simulink model "hex_recovery"  (R2025b)
settings: Solver=FixedStepDiscrete  StartTime=0.0  StopTime=P.duration  FixedStep=P.base_dt  RelTol=1e-3
model workspace (MAT data in the model file):
  P.mass = 3.4
  P.gravity = 9.81
  P.rotor_positions = [0.275  0  0; 0.1375  0.238156986041  0; -0.1375  0.238156986041  0; -0.275  3.36777869766e-17  0; -0.1375  -0.238156986041  0; 0.1375  -0.238156986041  0]
  P.J = [0.0305275  -2.60208521397e-18  0; -2.60208521397e-18  0.0305275  0; 0  0  0.059375]
  P.invJ = [32.7573499304  2.79215185988e-15  0; 2.79215185988e-15  32.7573499304  0; 0  0  16.8421052632]
  P.kT = [7.45e-06; 7.45e-06; 7.45e-06; 7.45e-06; 7.45e-06; 7.45e-06]
  P.kQ = [9.79675e-08; 9.79675e-08; 9.79675e-08; 9.79675e-08; 9.79675e-08; 9.79675e-08]
  P.yaw_sign = [1; -1; 1; -1; 1; -1]
  P.tau = [0.05; 0.05; 0.05; 0.05; 0.05; 0.05]
  P.omega_min = 0
  P.omega_max = 1100
  P.body_drag = [0.005; 0.005; 0.01]
  P.rotor_drag = [0.000119; 0.000119; 0.000232]
  P.A = [1  1  1  1  1  1; 0  0.238156986041  0.238156986041  3.36777869766e-17  -0.238156986041  -0.238156986041; -0.275  -0.1375  0.1375  0.275  0.1375  -0.1375; 0.01315  -0.01315  0.01315  -0.01315  0.01315  -0.01315]
  P.pinvA = [0.166666666667  -3.00435841323e-17  -1.21212121212  12.6742712294; 0.166666666667  1.04972776216  -0.606060606061  -12.6742712294; 0.166666666667  1.04972776216  0.606060606061  12.6742712294; 0.166666666667  1.03568818436e-16  1.21212121212  -12.6742712294; 0.166666666667  -1.04972776216  0.606060606061  12.6742712294; 0.166666666667  -1.04972776216  -0.606060606061  -12.6742712294]
  P.thrust_min = [0; 0; 0; 0; 0; 0]
  P.thrust_max = [9.0145; 9.0145; 9.0145; 9.0145; 9.0145; 9.0145]
  P.wrench_scale = [54.087; 8.58746460266; 9.91595; 0.71124405]
  P.row_weights = [0.0369774622368; 0.116448806053; 0.100847624282; 0.281197431458]
  P.regularization = 0
  P.control.yaw_hold_rad = 0
  P.control.position_p = [4; 4; 1.4]
  P.control.velocity_p = [7; 7; 3]
  P.control.velocity_i = [0.4; 0.4; 0.9]
  P.control.velocity_d = [0.1; 0.1; 0.1]
  P.control.attitude_p = [7; 7; 3]
  P.control.rate_p = [20; 20; 6]
  P.control.rate_i = [30; 30; 0.6]
  P.control.rate_d = [0.5; 0.5; 0.06]
  P.control.velocity_limit_m_s = [3; 3; 2]
  P.control.rate_limit_rad_s = [3; 3; 1.5]
  P.control.velocity_integral_limit_m_s2 = [2; 2; 2]
  P.control.rate_integral_limit_rad_s2 = [20; 20; 2]
  P.control.acceleration_limit_m_s2 = [4; 4; 4]
  P.control.tilt_limit_deg = 25
  P.control.derivative_filter_hz = 20
  P.control.antiwindup_gain_s_inv = 2
  P.control.recovery.estimator_tau_s = 0.025
  P.control.recovery.estimator_min_command_rad_s = 100
  P.control.recovery.failed_speed_ratio = 0.06
  P.control.recovery.healthy_speed_ratio = 0.98
  P.control.recovery.position_soft_m = 0.08
  P.control.recovery.position_hard_m = 0.3
  P.control.recovery.tilt_soft_deg = 12
  P.control.recovery.tilt_hard_deg = 25
  P.control.recovery.rate_soft_rad_s = 0.6
  P.control.recovery.rate_hard_rad_s = 2
  P.control.recovery.progress_slow_tau_s = 0.08
  P.control.recovery.progress_fast_tau_s = 0.8
  P.control.recovery.degraded_position_p = [1.5; 1.5; 1.4]
  P.control.recovery.degraded_velocity_p = [4; 4; 3]
  P.control.recovery.degraded_acceleration_limit_m_s2 = [1.5; 1.5; 3]
  P.control.recovery.degraded_tilt_limit_deg = 15
  P.control.recovery.yaw_damping_s_inv = 1
  P.control.recovery.degraded_wrench_priority = [6; 3; 3; 0.015]
  P.sensor.rate_hz = 100
  P.sensor.accel_noise_density = 0.0035
  P.sensor.gyro_noise_density = 0.0003
  P.sensor.accel_bias_diffusion = 0.002
  P.sensor.gyro_bias_diffusion = 2e-05
  P.sensor.additional_accel_sample_std = 0.008
  P.sensor.position_sample_std_m = 0.003
  P.sensor.velocity_sample_std_m_s = 0.01
  P.sensor.attitude_sample_std_rad = 0.0008
  P.sensor.rpm_sample_std_rad_s = 1
  P.sensor.lever_m = [0; 0; 0]
  P.sensor.installation_rotation_xyzw = [0; 0; 0; 1]
  P.sensor.feedback_delay_s = 0.01
  P.sensor.installation_matrix = [1  0  0; 0  1  0; 0  0  1]
  P.wind.mean_m_s = [0; 0; 0]
  P.wind.ou_stationary_std_m_s = 0.2
  P.wind.ou_correlation_time_s = 1
  P.wind.update_rate_hz = 100
  P.termination.position_norm_m = 25
  P.termination.speed_m_s = 20
  P.termination.body_rate_rad_s = 15
  P.termination.minimum_altitude_m = -2
  P.integration_dt = 0.002
  P.control_dt = 0.01
  P.sensor_dt = 0.01
  P.export_dt = 0.01
  P.base_dt = 0.01
  P.duration = 24
  P.reference_mode = 'recovery_path_progress'
  P.control_tuning_version = 'recovery_v3_20261023'
  P.initial_state = [0; 0; 2.5; 0; 0; 0; 0; 0; 0; 1; 0; 0; 0; 863.81392478; 863.81392478; 863.81392478; 863.81392478; 863.81392478; 863.81392478]
  P.task_family = 2
  P.task_origin = [0; 0; 2.5]
  P.motion_start = 1
  P.motion_end = 7
  P.heading = 0
  P.displacement = 1.2
  P.radius = 0.3
  P.turn = 6.28318530718
  P.fault_motor = 1
  P.fault_factor = 0
  P.fault_start = 3
  P.fault_end = Inf
  P.observed_feedback = 1
  P.noise_enabled = 1
  P.wind_enabled = 1
  P.feedback_delay = 0.03
  P.seed = 20261006
  P.external_force = [0; 0; 0]
  P.external_torque = [0; 0; 0]
  P.exogenous = [-0.419748102169 -0.416018697024 -0.42343299448 -0.41045202828 -0.394392977316 -0.434544678836 -0.402415922967 -0.400265397714 -0.40478587178 -0.425441360189 -0.422504362468 -0.40174926008 ... (57648 elements, 2402x24)]
  P_controller_step.control.yaw_hold_rad = 0
  P_controller_step.control.position_p = [4; 4; 1.4]
  P_controller_step.control.velocity_p = [7; 7; 3]
  P_controller_step.control.velocity_i = [0.4; 0.4; 0.9]
  P_controller_step.control.velocity_d = [0.1; 0.1; 0.1]
  P_controller_step.control.attitude_p = [7; 7; 3]
  P_controller_step.control.rate_p = [20; 20; 6]
  P_controller_step.control.rate_i = [30; 30; 0.6]
  P_controller_step.control.rate_d = [0.5; 0.5; 0.06]
  P_controller_step.control.velocity_limit_m_s = [3; 3; 2]
  P_controller_step.control.rate_limit_rad_s = [3; 3; 1.5]
  P_controller_step.control.velocity_integral_limit_m_s2 = [2; 2; 2]
  P_controller_step.control.rate_integral_limit_rad_s2 = [20; 20; 2]
  P_controller_step.control.acceleration_limit_m_s2 = [4; 4; 4]
  P_controller_step.control.tilt_limit_deg = 25
  P_controller_step.control.derivative_filter_hz = 20
  P_controller_step.control.antiwindup_gain_s_inv = 2
  P_controller_step.control.recovery.estimator_tau_s = 0.025
  P_controller_step.control.recovery.estimator_min_command_rad_s = 100
  P_controller_step.control.recovery.failed_speed_ratio = 0.06
  P_controller_step.control.recovery.healthy_speed_ratio = 0.98
  P_controller_step.control.recovery.position_soft_m = 0.08
  P_controller_step.control.recovery.position_hard_m = 0.3
  P_controller_step.control.recovery.tilt_soft_deg = 12
  P_controller_step.control.recovery.tilt_hard_deg = 25
  P_controller_step.control.recovery.rate_soft_rad_s = 0.6
  P_controller_step.control.recovery.rate_hard_rad_s = 2
  P_controller_step.control.recovery.progress_slow_tau_s = 0.08
  P_controller_step.control.recovery.progress_fast_tau_s = 0.8
  P_controller_step.control.recovery.degraded_position_p = [1.5; 1.5; 1.4]
  P_controller_step.control.recovery.degraded_velocity_p = [4; 4; 3]
  P_controller_step.control.recovery.degraded_acceleration_limit_m_s2 = [1.5; 1.5; 3]
  P_controller_step.control.recovery.degraded_tilt_limit_deg = 15
  P_controller_step.control.recovery.yaw_damping_s_inv = 1
  P_controller_step.control.recovery.degraded_wrench_priority = [6; 3; 3; 0.015]
  P_controller_step.control_dt = 0.01
  P_controller_step.mass = 3.4
  P_controller_step.gravity = 9.81
  P_controller_step.thrust_max = [9.0145; 9.0145; 9.0145; 9.0145; 9.0145; 9.0145]
  P_controller_step.J = [0.0305275  -2.60208521397e-18  0; -2.60208521397e-18  0.0305275  0; 0  0  0.059375]
  P_controller_step.kT = [7.45e-06; 7.45e-06; 7.45e-06; 7.45e-06; 7.45e-06; 7.45e-06]
  P_controller_step.A = [1  1  1  1  1  1; 0  0.238156986041  0.238156986041  3.36777869766e-17  -0.238156986041  -0.238156986041; -0.275  -0.1375  0.1375  0.275  0.1375  -0.1375; 0.01315  -0.01315  0.01315  -0.01315  0.01315  -0.01315]
  P_controller_step.pinvA = [0.166666666667  -3.00435841323e-17  -1.21212121212  12.6742712294; 0.166666666667  1.04972776216  -0.606060606061  -12.6742712294; 0.166666666667  1.04972776216  0.606060606061  12.6742712294; 0.166666666667  1.03568818436e-16  1.21212121212  -12.6742712294; 0.166666666667  -1.04972776216  0.606060606061  12.6742712294; 0.166666666667  -1.04972776216  -0.606060606061  -12.6742712294]
  P_controller_step.thrust_min = [0; 0; 0; 0; 0; 0]
  P_controller_step.row_weights = [0.0369774622368; 0.116448806053; 0.100847624282; 0.281197431458]
  P_controller_step.wrench_scale = [54.087; 8.58746460266; 9.91595; 0.71124405]
  P_controller_step.regularization = 0
  P_controller_step.tau = [0.05; 0.05; 0.05; 0.05; 0.05; 0.05]
  P_controller_step.omega_max = 1100
  P_controller_step.observed_feedback = 1
  P_controller_step.feedback_delay = 0.03
  P_controller_step.sensor_dt = 0.01
  P_envelope_step.termination.position_norm_m = 25
  P_envelope_step.termination.speed_m_s = 20
  P_envelope_step.termination.body_rate_rad_s = 15
  P_envelope_step.termination.minimum_altitude_m = -2
  P_fault_schedule.base_dt = 0.01
  P_fault_schedule.fault_start = 3
  P_fault_schedule.fault_end = Inf
  P_fault_schedule.fault_motor = 1
  P_fault_schedule.fault_factor = 0
  P_plant_step.rotor_positions = [0.275  0  0; 0.1375  0.238156986041  0; -0.1375  0.238156986041  0; -0.275  3.36777869766e-17  0; -0.1375  -0.238156986041  0; 0.1375  -0.238156986041  0]
  P_plant_step.rotor_drag = [0.000119; 0.000119; 0.000232]
  P_plant_step.kT = [7.45e-06; 7.45e-06; 7.45e-06; 7.45e-06; 7.45e-06; 7.45e-06]
  P_plant_step.kQ = [9.79675e-08; 9.79675e-08; 9.79675e-08; 9.79675e-08; 9.79675e-08; 9.79675e-08]
  P_plant_step.yaw_sign = [1; -1; 1; -1; 1; -1]
  P_plant_step.body_drag = [0.005; 0.005; 0.01]
  P_plant_step.gravity = 9.81
  P_plant_step.mass = 3.4
  P_plant_step.invJ = [32.7573499304  2.79215185988e-15  0; 2.79215185988e-15  32.7573499304  0; 0  0  16.8421052632]
  P_plant_step.J = [0.0305275  -2.60208521397e-18  0; -2.60208521397e-18  0.0305275  0; 0  0  0.059375]
  P_plant_step.tau = [0.05; 0.05; 0.05; 0.05; 0.05; 0.05]
  P_plant_step.integration_dt = 0.002
  P_sensor_step.rotor_positions = [0.275  0  0; 0.1375  0.238156986041  0; -0.1375  0.238156986041  0; -0.275  3.36777869766e-17  0; -0.1375  -0.238156986041  0; 0.1375  -0.238156986041  0]
  P_sensor_step.rotor_drag = [0.000119; 0.000119; 0.000232]
  P_sensor_step.kT = [7.45e-06; 7.45e-06; 7.45e-06; 7.45e-06; 7.45e-06; 7.45e-06]
  P_sensor_step.kQ = [9.79675e-08; 9.79675e-08; 9.79675e-08; 9.79675e-08; 9.79675e-08; 9.79675e-08]
  P_sensor_step.yaw_sign = [1; -1; 1; -1; 1; -1]
  P_sensor_step.body_drag = [0.005; 0.005; 0.01]
  P_sensor_step.gravity = 9.81
  P_sensor_step.mass = 3.4
  P_sensor_step.invJ = [32.7573499304  2.79215185988e-15  0; 2.79215185988e-15  32.7573499304  0; 0  0  16.8421052632]
  P_sensor_step.J = [0.0305275  -2.60208521397e-18  0; -2.60208521397e-18  0.0305275  0; 0  0  0.059375]
  P_sensor_step.tau = [0.05; 0.05; 0.05; 0.05; 0.05; 0.05]
  P_sensor_step.sensor.rate_hz = 100
  P_sensor_step.sensor.accel_noise_density = 0.0035
  P_sensor_step.sensor.gyro_noise_density = 0.0003
  P_sensor_step.sensor.accel_bias_diffusion = 0.002
  P_sensor_step.sensor.gyro_bias_diffusion = 2e-05
  P_sensor_step.sensor.additional_accel_sample_std = 0.008
  P_sensor_step.sensor.position_sample_std_m = 0.003
  P_sensor_step.sensor.velocity_sample_std_m_s = 0.01
  P_sensor_step.sensor.attitude_sample_std_rad = 0.0008
  P_sensor_step.sensor.rpm_sample_std_rad_s = 1
  P_sensor_step.sensor.lever_m = [0; 0; 0]
  P_sensor_step.sensor.installation_rotation_xyzw = [0; 0; 0; 1]
  P_sensor_step.sensor.feedback_delay_s = 0.01
  P_sensor_step.sensor.installation_matrix = [1  0  0; 0  1  0; 0  0  1]
  P_sensor_step.sensor_dt = 0.01
  P_sensor_step.exogenous = [-0.419748102169 -0.416018697024 -0.42343299448 -0.41045202828 -0.394392977316 -0.434544678836 -0.402415922967 -0.400265397714 -0.40478587178 -0.425441360189 -0.422504362468 -0.40174926008 ... (57648 elements, 2402x24)]
  P_sensor_step.noise_enabled = 1
  P_sensor_step.observed_feedback = 1
  P_sensor_step.feedback_delay = 0.03
  P_task_reference.task_origin = [0; 0; 2.5]
  P_task_reference.task_family = 2
  P_task_reference.motion_start = 1
  P_task_reference.motion_end = 7
  P_task_reference.heading = 0
  P_task_reference.displacement = 1.2
  P_task_reference.radius = 0.3
  P_task_reference.turn = 6.28318530718
  P_task_reference.control.yaw_hold_rad = 0
  P_task_reference.control.position_p = [4; 4; 1.4]
  P_task_reference.control.velocity_p = [7; 7; 3]
  P_task_reference.control.velocity_i = [0.4; 0.4; 0.9]
  P_task_reference.control.velocity_d = [0.1; 0.1; 0.1]
  P_task_reference.control.attitude_p = [7; 7; 3]
  P_task_reference.control.rate_p = [20; 20; 6]
  P_task_reference.control.rate_i = [30; 30; 0.6]
  P_task_reference.control.rate_d = [0.5; 0.5; 0.06]
  P_task_reference.control.velocity_limit_m_s = [3; 3; 2]
  P_task_reference.control.rate_limit_rad_s = [3; 3; 1.5]
  P_task_reference.control.velocity_integral_limit_m_s2 = [2; 2; 2]
  P_task_reference.control.rate_integral_limit_rad_s2 = [20; 20; 2]
  P_task_reference.control.acceleration_limit_m_s2 = [4; 4; 4]
  P_task_reference.control.tilt_limit_deg = 25
  P_task_reference.control.derivative_filter_hz = 20
  P_task_reference.control.antiwindup_gain_s_inv = 2
  P_task_reference.control.recovery.estimator_tau_s = 0.025
  P_task_reference.control.recovery.estimator_min_command_rad_s = 100
  P_task_reference.control.recovery.failed_speed_ratio = 0.06
  P_task_reference.control.recovery.healthy_speed_ratio = 0.98
  P_task_reference.control.recovery.position_soft_m = 0.08
  P_task_reference.control.recovery.position_hard_m = 0.3
  P_task_reference.control.recovery.tilt_soft_deg = 12
  P_task_reference.control.recovery.tilt_hard_deg = 25
  P_task_reference.control.recovery.rate_soft_rad_s = 0.6
  P_task_reference.control.recovery.rate_hard_rad_s = 2
  P_task_reference.control.recovery.progress_slow_tau_s = 0.08
  P_task_reference.control.recovery.progress_fast_tau_s = 0.8
  P_task_reference.control.recovery.degraded_position_p = [1.5; 1.5; 1.4]
  P_task_reference.control.recovery.degraded_velocity_p = [4; 4; 3]
  P_task_reference.control.recovery.degraded_acceleration_limit_m_s2 = [1.5; 1.5; 3]
  P_task_reference.control.recovery.degraded_tilt_limit_deg = 15
  P_task_reference.control.recovery.yaw_damping_s_inv = 1
  P_task_reference.control.recovery.degraded_wrench_priority = [6; 3; 3; 0.015]
  P_task_reference.control_dt = 0.01
  P_wind_step.sensor_dt = 0.01
  P_wind_step.exogenous = [-0.419748102169 -0.416018697024 -0.42343299448 -0.41045202828 -0.394392977316 -0.434544678836 -0.402415922967 -0.400265397714 -0.40478587178 -0.425441360189 -0.422504362468 -0.40174926008 ... (57648 elements, 2402x24)]
  P_wind_step.wind_enabled = 1
  P_wind_step.external_force = [0; 0; 0]
  P_wind_step.external_torque = [0; 0; 0]
values from neighbouring files (symbols this model uses):
  P = hex_recovery_parameters(); ws.assignin('P',P)    [build_hex_recovery_model.m]    (also in diagnose_hex_healthy_tilt.m = base.parameters; hex_recovery_metrics.m = result.parameters; hex_recovery_parameters.m = hex_prepare_inputs(P); my_simulation.m = hex_prepare_inputs(P))
Description:
  | Six-rotor research simulation migrated from a6b9f1dd3d839416e469755490b8ff7733acd4ee. ENU world, FLU body, Hamilton xyzw, SI units. Embedded MATLAB Function code; no Python runtime. 100 Hz controller/sensors, 500 Hz RK4 substeps; fault truth enters plant only.
  | 
  | # SciPy trust-region-reflective algorithm
  | 
  | `functions/hex_trf.m` is a MATLAB translation/adaptation of the bounded linear least-squares algorithm in SciPy 1.17.1:
  | 
  | - `scipy/optimize/_lsq/trf_linear.py`
  | - `scipy/optimize/_lsq/common.py` (bounded-linear-solver helpers)
  | - `scipy/optimize/_lsq/givens_elimination.pyx`
  | 
  | Source: https://github.com/scipy/scipy/tree/v1.17.1/scipy/optimize/_lsq
  | 
  | The implementation is restricted to six variables with finite bounds and uses MATLAB's QR/SVD kernels. It is embedded in the delivered SLX; the upstream Python runtime and SciPy binaries are not required for simulation.
  | 
  | ```text
  | Copyright (c) 2001-2002 Enthought, Inc. 2003, SciPy Developers.
  | All rights reserved.
  | 
  | Redistribution and use in source and binary forms, with or without
  | modification, are permitted provided that the following conditions
  | are met:
  | 
  | 1. Redistributions of source code must retain the above copyright
  |    notice, this list of conditions and the following disclaimer.
  | 
  | 2. Redistributions in binary form must reproduce the above
  |    copyright notice, this list of conditions and the following
  |    disclaimer in the documentation and/or other materials provided
  |    with the distribution.
  | 
  | 3. Neither the name of the copyright holder nor the names of its
  |    contributors may be used to endorse or promote products derived
  |    from this software without specific prior written permission.
  | 
  | THIS SOFTWARE IS PROVIDED BY THE COPYRIGHT HOLDERS AND CONTRIBUTORS
  | "AS IS" AND ANY EXPRESS OR IMPLIED WARRANTIES, INCLUDING, BUT NOT
  | LIMITED TO, THE IMPLIED WARRANTIES OF MERCHANTABILITY AND FITNESS FOR
  | A PARTICULAR PURPOSE ARE DISCLAIMED. IN NO EVENT SHALL THE COPYRIGHT
  | OWNER OR CONTRIBUTORS BE LIABLE FOR ANY DIRECT, INDIRECT, INCIDENTAL,
  | SPECIAL, EXEMPLARY, OR CONSEQUENTIAL DAMAGES (INCLUDING, BUT NOT
  | LIMITED TO, PROCUREMENT OF SUBSTITUTE GOODS OR SERVICES; LOSS OF USE,
  | DATA, OR PROFITS; OR BUSINESS INTERRUPTION) HOWEVER CAUSED AND ON ANY
  | THEORY OF LIABILITY, WHETHER IN CONTRACT, STRICT LIABILITY, OR TORT
  | (INCLUDING NEGLIGENCE OR OTHERWISE) ARISING IN ANY WAY OUT OF THE USE
  | OF THIS SOFTWARE, EVEN IF ADVISED OF THE POSSIBILITY OF SUCH DAMAGE.
  | ```
  | 
  | 
  | Copyright 2023 RotorPy Authors
  | 
  | Permission is hereby granted, free of charge, to any person obtaining a copy of this software and associated documentation files (the "Software"), to deal in the Software without restriction, including without limitation the rights to use, copy, modify, merge, publish, distribute, sublicense, and/or sell copies of the Software, and to permit persons to whom the Software is furnished to do so, subject to the following conditions:
  | 
  | The above copyright notice and this permission notice shall be included in all copies or substantial portions of the Software.
  | 
  | THE SOFTWARE IS PROVIDED "AS IS", WITHOUT WARRANTY OF ANY KIND, EXPRESS OR IMPLIED, INCLUDING BUT NOT LIMITED TO THE WARRANTIES OF MERCHANTABILITY, FITNESS FOR A PARTICULAR PURPOSE AND NONINFRINGEMENT. IN NO EVENT SHALL THE AUTHORS OR COPYRIGHT HOLDERS BE LIABLE FOR ANY CLAIM, DAMAGES OR OTHER LIABILITY, WHETHER IN AN ACTION OF CONTRACT, TORT OR OTHERWISE, ARISING FROM, OUT OF OR IN CONNECTION WITH THE SOFTWARE OR THE USE OR OTHER DEALINGS IN THE SOFTWARE.
  | 
  | PV reference: position/velocity only; internal fixed heading; no acceleration or yaw-rate feedforward.
  | Recovery experiment 2026-10-23: RPM-based estimate; thrust-direction priority; measured-state path retiming.
settings Model: Creator=lenovo  LastModifiedBy=lenovo
settings DataIOCC: SaveOutput=off  SignalLogging=off

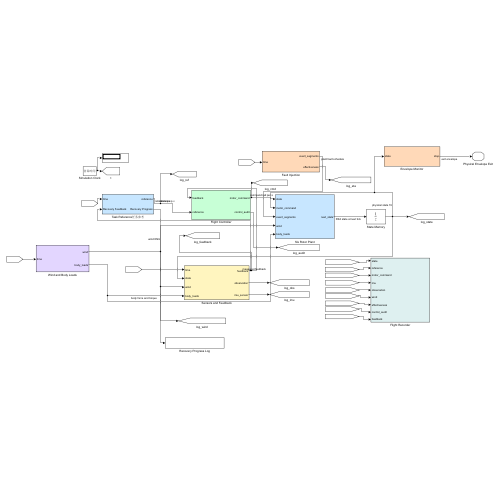
[thumbnail: Simulink's stored preview of the top-level diagram]
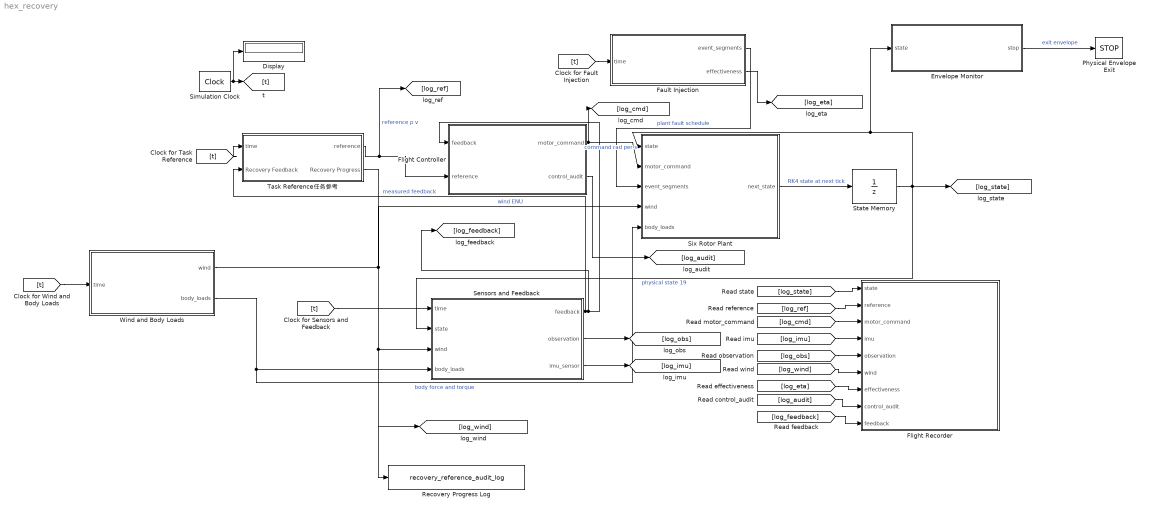
== system hex_recovery ==
  Display : Display
  Envelope Monitor : Subsystem
  Fault Injection : Subsystem
  Flight Controller : Subsystem
  Flight Recorder : Subsystem
  Physical Envelope Exit : Stop
  Recovery Progress Log : ToWorkspace  VariableName=recovery_reference_audit_log  SaveFormat=Timeseries  SampleTime=P.export_dt
  Sensors and Feedback : Subsystem
  Simulation Clock : DigitalClock  SampleTime=P.base_dt
      mask DialogControl ParameterGroupVar Prompt: 参数
      mask Display: disp('仿真时间')
  Six Rotor Plant : Subsystem
  State Memory : UnitDelay  InitialCondition=P.initial_state  SampleTime=P.base_dt  HasFrameUpgradeWarning=on
  Task Reference任务参考 : Subsystem
  Wind and Body Loads : Subsystem
  wires:
  Simulation Clock/1 -> Display/1, [t]
  [t] -> Task Reference任务参考/1(time)
  [t] -> Fault Injection/1(time)
  [t] -> Wind and Body Loads/1(time)
  [t] -> Sensors and Feedback/1(time)
  Task Reference任务参考/1(reference) -> Flight Controller/2(reference), [log_ref]  "reference p v"
  Sensors and Feedback/1(feedback) -> Flight Controller/1(feedback), [log_feedback], Task Reference任务参考/2(Recovery Feedback)  "measured feedback"
  Flight Controller/1(motor_command) -> Six Rotor Plant/2(motor_command), [log_cmd]  "command rad per s"
  Fault Injection/1(event_segments) -> Six Rotor Plant/3(event_segments)  "plant fault schedule"
  Wind and Body Loads/1(wind) -> Sensors and Feedback/3(wind), [log_wind], Six Rotor Plant/4(wind)  "wind ENU"
  Wind and Body Loads/2(body_loads) -> Sensors and Feedback/4(body_loads), Six Rotor Plant/5(body_loads)  "body force and torque"
  Six Rotor Plant/1(next_state) -> State Memory/1  "RK4 state at next tick"
  State Memory/1 -> Six Rotor Plant/1(state), Envelope Monitor/1(state), [log_state], Sensors and Feedback/2(state)  "physical state 19"
  Envelope Monitor/1(stop) -> Physical Envelope Exit/1  "exit envelope"
  [log_state] -> Flight Recorder/1(state)
  [log_ref] -> Flight Recorder/2(reference)
  [log_cmd] -> Flight Recorder/3(motor_command)
  Sensors and Feedback/3(imu_sensor) -> [log_imu]
  [log_imu] -> Flight Recorder/4(imu)
  Sensors and Feedback/2(observation) -> [log_obs]
  [log_obs] -> Flight Recorder/5(observation)
  [log_wind] -> Flight Recorder/6(wind)
  Fault Injection/2(effectiveness) -> [log_eta]
  [log_eta] -> Flight Recorder/7(effectiveness)
  Flight Controller/2(control_audit) -> [log_audit]
  [log_audit] -> Flight Recorder/8(control_audit)
  [log_feedback] -> Flight Recorder/9(feedback)
  Task Reference任务参考/2(Recovery Progress) -> Recovery Progress Log/1

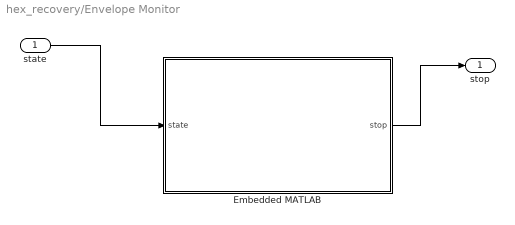
== system hex_recovery/Envelope Monitor ==
  state : Inport
  Embedded MATLAB : MATLAB Function  TreatAsAtomicUnit=on
  stop : Outport
  wires:
  state/1 -> Embedded MATLAB/1(state)
  Embedded MATLAB/1(stop) -> stop/1

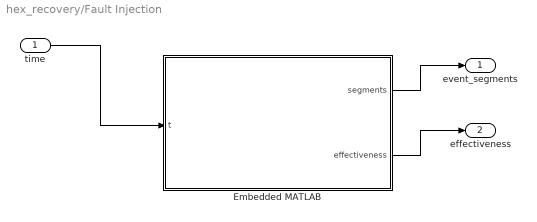
== system hex_recovery/Fault Injection ==
  time : Inport
  Embedded MATLAB : MATLAB Function  TreatAsAtomicUnit=on
  event_segments : Outport
  effectiveness : Outport  Port=2
  wires:
  time/1 -> Embedded MATLAB/1(t)
  Embedded MATLAB/1(segments) -> event_segments/1
  Embedded MATLAB/2(effectiveness) -> effectiveness/1

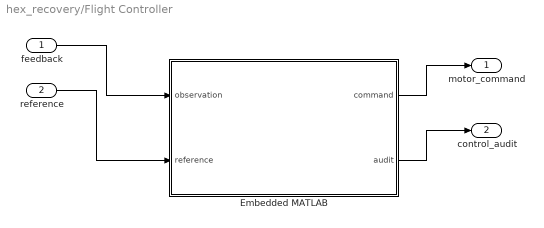
== system hex_recovery/Flight Controller ==
  feedback : Inport
  reference : Inport  Port=2
  Embedded MATLAB : MATLAB Function  TreatAsAtomicUnit=on
  motor_command : Outport
  control_audit : Outport  Port=2
  wires:
  feedback/1 -> Embedded MATLAB/1(observation)
  reference/1 -> Embedded MATLAB/2(reference)
  Embedded MATLAB/1(command) -> motor_command/1
  Embedded MATLAB/2(audit) -> control_audit/1

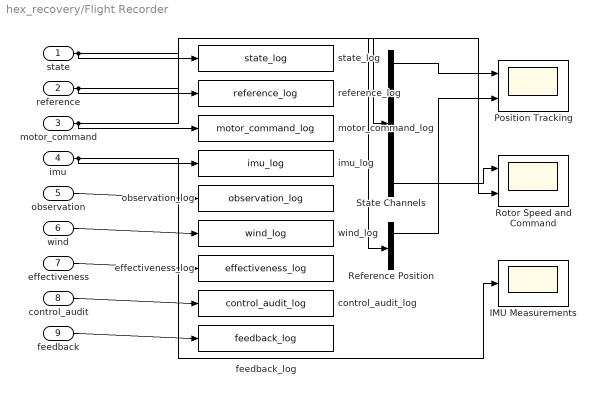
== system hex_recovery/Flight Recorder ==
  state : Inport
  reference : Inport  Port=2
  motor_command : Inport  Port=3
  imu : Inport  Port=4
  observation : Inport  Port=5
  wind : Inport  Port=6
  effectiveness : Inport  Port=7
  control_audit : Inport  Port=8
  feedback : Inport  Port=9
  IMU Measurements : Scope
  Position Tracking : Scope  NumInputPorts=2
  Reference Position : Demux  Outputs=[3 3]
  Rotor Speed and Command : Scope  NumInputPorts=2
  State Channels : Demux  Outputs=[3 3 4 3 6]
  control_audit_log : ToWorkspace  VariableName=control_audit_log  SaveFormat=Timeseries  SampleTime=P.export_dt
  effectiveness_log : ToWorkspace  VariableName=effectiveness_log  SaveFormat=Timeseries  SampleTime=P.export_dt
  feedback_log : ToWorkspace  VariableName=feedback_log  SaveFormat=Timeseries  SampleTime=P.export_dt
  imu_log : ToWorkspace  VariableName=imu_log  SaveFormat=Timeseries  SampleTime=P.export_dt
  motor_command_log : ToWorkspace  VariableName=motor_command_log  SaveFormat=Timeseries  SampleTime=P.export_dt
  observation_log : ToWorkspace  VariableName=observation_log  SaveFormat=Timeseries  SampleTime=P.export_dt
  reference_log : ToWorkspace  VariableName=reference_log  SaveFormat=Timeseries  SampleTime=P.export_dt
  state_log : ToWorkspace  VariableName=state_log  SaveFormat=Timeseries  SampleTime=P.export_dt
  wind_log : ToWorkspace  VariableName=wind_log  SaveFormat=Timeseries  SampleTime=P.export_dt
  wires:
  state/1 -> state_log/1, State Channels/1
  reference/1 -> reference_log/1, Reference Position/1
  motor_command/1 -> motor_command_log/1, Rotor Speed and Command/2
  imu/1 -> imu_log/1, IMU Measurements/1
  observation/1 -> observation_log/1
  wind/1 -> wind_log/1
  effectiveness/1 -> effectiveness_log/1
  control_audit/1 -> control_audit_log/1
  feedback/1 -> feedback_log/1
  State Channels/1 -> Position Tracking/1
  Reference Position/1 -> Position Tracking/2
  State Channels/5 -> Rotor Speed and Command/1

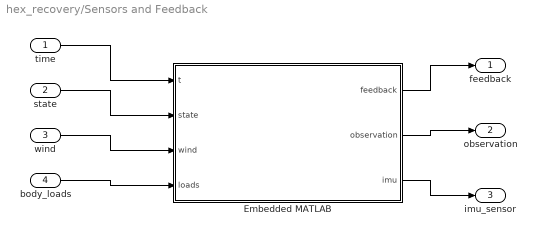
== system hex_recovery/Sensors and Feedback ==
  time : Inport
  state : Inport  Port=2
  wind : Inport  Port=3
  body_loads : Inport  Port=4
  Embedded MATLAB : MATLAB Function  TreatAsAtomicUnit=on
  feedback : Outport
  observation : Outport  Port=2
  imu_sensor : Outport  Port=3
  wires:
  time/1 -> Embedded MATLAB/1(t)
  state/1 -> Embedded MATLAB/2(state)
  wind/1 -> Embedded MATLAB/3(wind)
  body_loads/1 -> Embedded MATLAB/4(loads)
  Embedded MATLAB/1(feedback) -> feedback/1
  Embedded MATLAB/2(observation) -> observation/1
  Embedded MATLAB/3(imu) -> imu_sensor/1

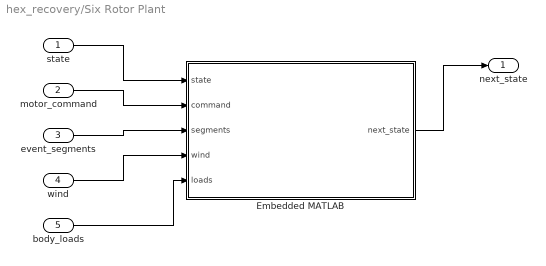
== system hex_recovery/Six Rotor Plant ==
  state : Inport
  motor_command : Inport  Port=2
  event_segments : Inport  Port=3
  wind : Inport  Port=4
  body_loads : Inport  Port=5
  Embedded MATLAB : MATLAB Function  TreatAsAtomicUnit=on
  next_state : Outport
  wires:
  state/1 -> Embedded MATLAB/1(state)
  motor_command/1 -> Embedded MATLAB/2(command)
  event_segments/1 -> Embedded MATLAB/3(segments)
  wind/1 -> Embedded MATLAB/4(wind)
  body_loads/1 -> Embedded MATLAB/5(loads)
  Embedded MATLAB/1(next_state) -> next_state/1

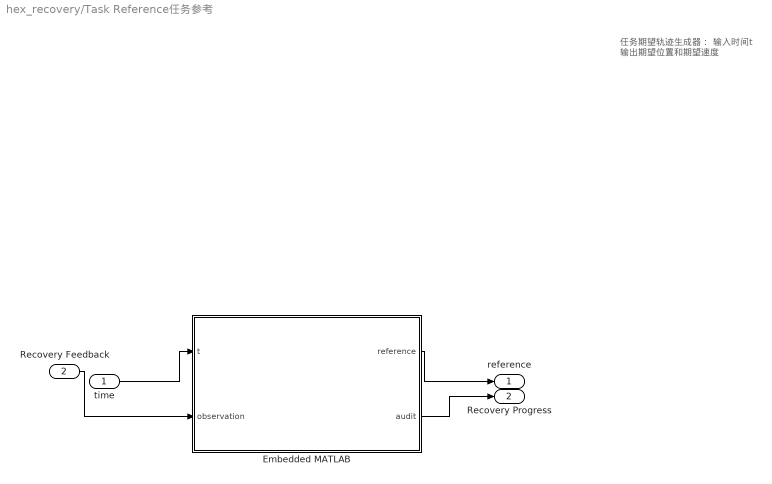
== system hex_recovery/Task Reference任务参考 ==
  note: 任务期望轨迹生成器：
      | 输入时间t
      | 输出期望位置和期望速度
  time : Inport
  Recovery Feedback : Inport  Port=2
  Embedded MATLAB : MATLAB Function  TreatAsAtomicUnit=on
  reference : Outport
  Recovery Progress : Outport  Port=2
  wires:
  time/1 -> Embedded MATLAB/1(t)
  Embedded MATLAB/1(reference) -> reference/1
  Recovery Feedback/1 -> Embedded MATLAB/2(observation)
  Embedded MATLAB/2(audit) -> Recovery Progress/1

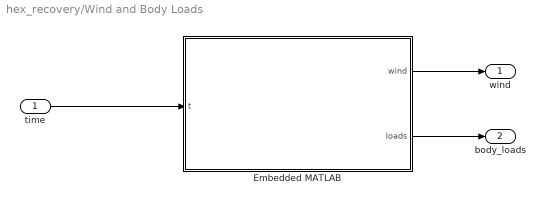
== system hex_recovery/Wind and Body Loads ==
  time : Inport
  Embedded MATLAB : MATLAB Function  TreatAsAtomicUnit=on
  wind : Outport
  body_loads : Outport  Port=2
  wires:
  time/1 -> Embedded MATLAB/1(t)
  Embedded MATLAB/1(wind) -> wind/1
  Embedded MATLAB/2(loads) -> body_loads/1

== matlab function hex_recovery/Flight Controller/Embedded MATLAB ==
  settings: updateMethod=DISCRETE  sampleTime=P.control_dt
  data: observation input; command output; reference input; audit output; P_controller_step parameter
function [command,audit]=recovery_controller_step(observation,reference,P_controller_step)
%#codegen
% Motor response is estimated from RPM feedback and delayed command history.
% Fault truth is not an input. eta_hat describes command-to-thrust loss only
% for this project's first-order motor-target failure model.
persistent previous_w previous_v filtered_alpha filtered_accel vi ri last_qd
persistent previous_rpm speed_ratio command_history ticks initialized
if isempty(initialized)
    previous_w=zeros(3,1); previous_v=zeros(3,1);
    filtered_alpha=zeros(3,1); filtered_accel=zeros(3,1);
    vi=zeros(3,1); ri=zeros(3,1); last_qd=[0;0;0;1];
    previous_rpm=zeros(6,1); speed_ratio=ones(6,1);
    command_history=zeros(6,1001); ticks=0; initialized=false;
end
x=observation(1:3); v=observation(4:6);
q=observation(7:10); q=q/norm(q); w=observation(11:13);
rpm=observation(14:19); R=hex_rotation(q);
c=P_controller_step.control; r=c.recovery; dt=P_controller_step.control_dt;
delay_ticks=0;
if P_controller_step.observed_feedback, delay_ticks=ceil(P_controller_step.feedback_delay/P_controller_step.sensor_dt-1e-10); end
if initialized && ticks>delay_ticks
    previous_command=command_history(:,mod(ticks-delay_ticks-1,1001)+1);
    decay=exp(-dt./P_controller_step.tau);
    for i=1:6
        if previous_command(i)>=r.estimator_min_command_rad_s
            observed=(rpm(i)-decay(i)*previous_rpm(i))/...
                ((1-decay(i))*previous_command(i));
            observed=min(max(observed,0),1.1);
            speed_ratio(i)=speed_ratio(i)+(1-exp(-dt/r.estimator_tau_s))*(observed-speed_ratio(i));
        end
    end
end
eta=min(speed_ratio.^2,1);
eta(speed_ratio>=r.healthy_speed_ratio)=1;
eta(speed_ratio<r.failed_speed_ratio)=0;
damage=min(max((1-min(eta))/.8,0),1);
position_p=(1-damage)*c.position_p+damage*r.degraded_position_p;
velocity_p=(1-damage)*c.velocity_p+damage*r.degraded_velocity_p;
acc_limit=(1-damage)*c.acceleration_limit_m_s2+damage*r.degraded_acceleration_limit_m_s2;
tilt_limit=(1-damage)*c.tilt_limit_deg+damage*r.degraded_tilt_limit_deg;
vi_applied=vi; ri_applied=ri;
ev=min(max(reference(4:6)+position_p.*(reference(1:3)-x),...
    -c.velocity_limit_m_s),c.velocity_limit_m_s)-v;
filt=1-exp(-2*pi*c.derivative_filter_hz*dt);
if initialized
    filtered_alpha=filtered_alpha+filt*((w-previous_w)/dt-filtered_alpha);
    filtered_accel=filtered_accel+filt*((v-previous_v)/dt-filtered_accel);
end
a_raw=velocity_p.*ev+vi-c.velocity_d.*filtered_accel;
acc=min(max(a_raw,-acc_limit),acc_limit);
F=P_controller_step.mass*(acc+[0;0;P_controller_step.gravity]); F(3)=max(F(3),0);
max_horizontal=F(3)*tan(tilt_limit*pi/180);
if norm(F(1:2))>max_horizontal
    F(1:2)=F(1:2)*max_horizontal/max(norm(F(1:2)),1e-12);
end
maximum=sum(eta.*P_controller_step.thrust_max);
if norm(F)>maximum, F=F*maximum/max(norm(F),1e-12); end
qd=hex_desired_attitude(F,c.yaw_hold_rad,last_qd);
e=hex_multiply([-q(1:3);q(4)],qd);
sgn=1; if e(4)<0, sgn=-1; end
attitude_error=2*sgn*e(1:3);
if damage>.1
    % Thrust direction has priority over heading during degraded flight.
    attitude_error=R'*cross(R(:,3),F/max(norm(F),1e-12));
end
rates=min(max(c.attitude_p.*attitude_error,-c.rate_limit_rad_s),c.rate_limit_rad_s);
error=rates-w;
alpha=c.rate_p.*error+ri-c.rate_d.*filtered_alpha;
if damage>.1
    rates(3)=0; error(3)=-w(3);
    alpha(3)=-r.yaw_damping_s_inv*w(3); ri(3)=0;
end
moment=P_controller_step.J*alpha+cross(w,P_controller_step.J*w);
desired=[max(F'*R(:,3),0);moment];
Q=P_controller_step; Q.thrust_max=max(eta.*P_controller_step.thrust_max,1e-9);
Q.thrust_min=zeros(6,1);
if damage>.1, Q.row_weights=r.degraded_wrench_priority./P_controller_step.wrench_scale; end
[thrust,residual,flags]=hex_allocate(desired,Q);
thrust=min(thrust,eta.*P_controller_step.thrust_max);
di=c.rate_i.*error*dt; di((residual(2:4).*error)>1e-8)=0;
if damage>.1, di(3)=0; end
ri=min(max(ri+di,-c.rate_integral_limit_rad_s2),c.rate_integral_limit_rad_s2);
limited_acc=F/P_controller_step.mass-[0;0;P_controller_step.gravity]; direction=F/max(norm(F),1e-12);
vi=min(max(vi+dt*(c.velocity_i.*ev+c.antiwindup_gain_s_inv*...
    (limited_acc-a_raw-direction*residual(1)/P_controller_step.mass)),...
    -c.velocity_integral_limit_m_s2),c.velocity_integral_limit_m_s2);
command=min(sqrt(max(thrust,0)./P_controller_step.kT)./max(sqrt(eta),1e-8),P_controller_step.omega_max);
command(eta==0)=0;
audit=[desired;P_controller_step.A*thrust;residual;vi;ri;reference(1:3)-x;ev;error;qd;rates;flags;...
    vi_applied;ri_applied;eta;damage];
command_history(:,mod(ticks,1001)+1)=command;
previous_rpm=rpm; previous_w=w; previous_v=v; last_qd=qd;
ticks=ticks+1; initialized=true;
end

function R=hex_rotation(q)
q=q/norm(q); v=q(1:3); w=q(4);
S=[0 -v(3) v(2);v(3) 0 -v(1);-v(2) v(1) 0];
R=eye(3)+2*w*S+2*S*S;
end

function q=hex_multiply(a,b)
q=[a(4)*b(1:3)+b(4)*a(1:3)+cross(a(1:3),b(1:3));a(4)*b(4)-a(1:3)'*b(1:3)];
end

function q=hex_desired_attitude(F,yaw,previous)
if norm(F)<1e-10
    q=previous/norm(previous); return
end
z=F/norm(F); y=cross(z,[cos(yaw);sin(yaw);0]);
if norm(y)<1e-10
    [~,i]=min(abs(z)); basis=zeros(3,1); basis(i)=1; y=cross(z,basis);
end
y=y/norm(y); x=cross(y,z); R=[x,y,z];
% Hamilton xyzw; branch on the largest component for numerical stability.
choices=[R(1,1);R(2,2);R(3,3);trace(R)]; [~,i]=max(choices);
if i==4
    w=sqrt(max(0,1+trace(R)))/2;
    q=[(R(3,2)-R(2,3))/(4*w);(R(1,3)-R(3,1))/(4*w);(R(2,1)-R(1,2))/(4*w);w];
else
    j=mod(i,3)+1; k=mod(j,3)+1;
    q=zeros(4,1); q(i)=sqrt(max(0,1+R(i,i)-R(j,j)-R(k,k)))/2;
    q(j)=(R(j,i)+R(i,j))/(4*q(i)); q(k)=(R(k,i)+R(i,k))/(4*q(i));
    q(4)=(R(k,j)-R(j,k))/(4*q(i));
end
q=q/norm(q);
end

function [thrust,residual,flags]=hex_allocate(desired,P_controller_step)
candidate=P_controller_step.pinvA*desired;
if P_controller_step.regularization==0 && all(candidate>=P_controller_step.thrust_min-1e-8) && all(candidate<=P_controller_step.thrust_max+1e-8) && norm(P_controller_step.row_weights.*(desired-P_controller_step.A*candidate))<=1e-10
    thrust=min(max(candidate,P_controller_step.thrust_min),P_controller_step.thrust_max); success=true;
else
    weights=diag(P_controller_step.row_weights);
    C=[weights*P_controller_step.A;sqrt(P_controller_step.regularization)*diag(1./max(P_controller_step.thrust_max-P_controller_step.thrust_min,1e-12))];
    d=[weights*desired;zeros(6,1)];
    [thrust,exitflag]=hex_trf(C,d,P_controller_step.thrust_min,P_controller_step.thrust_max);
    thrust=min(max(thrust,P_controller_step.thrust_min),P_controller_step.thrust_max);
    % A rank-deficient six-actuator problem can return a nonpositive flag
    % after reaching its optimum. Independently verify convex box KKT terms.
    gradient=C'*(C*thrust-d);
    projected=gradient;
    at_lower=thrust<=P_controller_step.thrust_min+1e-8;
    at_upper=thrust>=P_controller_step.thrust_max-1e-8;
    projected(at_lower)=min(gradient(at_lower),0);
    projected(at_upper)=max(gradient(at_upper),0);
    success=all(isfinite(thrust)) && (exitflag>0 || norm(projected,Inf)<=1e-10);
    if ~success
        fprintf('ALLOCATION_FAILURE flag=%g kkt=%.17g desired=[%.17g %.17g %.17g %.17g]\n',exitflag,norm(projected,Inf),desired(1),desired(2),desired(3),desired(4));
    end
end
residual=desired-P_controller_step.A*thrust;
boundtol=max(1e-8,1e-7*max(1,P_controller_step.thrust_max-P_controller_step.thrust_min));
active=(abs(thrust-P_controller_step.thrust_min)<=boundtol)|(abs(thrust-P_controller_step.thrust_max)<=boundtol);
flags=[double(success);sum(active);double(max(abs(residual./P_controller_step.wrench_scale))<=1e-6)];
assert(success,'Nominal allocation failed to converge.');
end

function [x,status]=hex_trf(A,b,lb,ub)
%HEX_TRF Six-variable trust-region-reflective bounded linear least squares.
% Algorithm translated from scipy.optimize._lsq.trf_linear/common, SciPy
% 1.17.1 (BSD-3-Clause; see THIRD_PARTY_NOTICES.md).
tol=1e-10;
QT=zeros(6,10); Rbase=zeros(6,6);
if all(A(5:10,:)==0,'all')
    x=pinv(A(1:4,:))*b(1:4);
    [Qsmall,Rsmall,E]=qr(A(1:4,:));
    QT(1:4,1:4)=Qsmall'; Rbase(1:4,:)=Rsmall;
else
    x=pinv(A)*b;
    [Qfull,Rfull,E]=qr(A,'econ'); QT=Qfull'; Rbase=Rfull;
end
[~,permutation]=max(E,[],1);
if all(x>=lb) && all(x<=ub), status=3; return; end
x=interior(reflect(x,lb,ub),lb,ub,.1);
r=A*x-b; g=A'*r; cost=.5*(r'*r); status=0;
for iteration=1:200
    v=ones(6,1); dv=zeros(6,1);
    for j=1:6
        if g(j)<0, v(j)=ub(j)-x(j); dv(j)=-1;
        elseif g(j)>0, v(j)=x(j)-lb(j); dv(j)=1;
        end
    end
    gnorm=norm(g.*v,Inf);
    if gnorm<tol, status=1; end
    if status~=0, break; end
    h=g.*dv; d=sqrt(v); gh=d.*g; Ah=A.*d';
    ph=-regularized_qr(Rbase.*d(permutation)',QT*r,permutation,sqrt(h));
    p=d.*ph; pg=p'*g;
    if pg>0, status=-1; end
    theta=1-min(.005,gnorm);
    step=select_step(x,Ah,gh,h,p,ph,d,lb,ub,theta);
    change=-quadratic(A,g,step,zeros(6,1));
    if change<0
        alpha=1;
        for backtrack=1:100
            xn=reflect(x+alpha*p,lb,ub); step=xn-x;
            change=-quadratic(A,g,step,zeros(6,1));
            if change>-.1*alpha*pg, break; end
            alpha=alpha*.5;
        end
        if any(active_bounds(xn,lb,ub,1e-10)~=0)
            xn=interior(reflect(x+theta*alpha*p,lb,ub),lb,ub,0);
            step=xn-x; change=-quadratic(A,g,step,zeros(6,1));
        end
        % Preserve the upstream backtracking routine's returned x exactly.
    else
        x=interior(x+step,lb,ub,0);
    end
    r=A*x-b; g=A'*r;
    if change<tol*cost, status=2; end
    cost=.5*(r'*r);
end
end

function x=regularized_qr(R,rhs,permutation,diagonal)
diagonal=diagonal(permutation);
for i=1:6
    if diagonal(i)==0, continue; end
    row=zeros(6,1); row(i)=diagonal(i); u=0;
    for j=i:6
        if row(j)~=0
            f=R(j,j); g=row(j);
            if f==0
                cs=0; sn=sign(g); radius=abs(g);
            else
                radius=sign(f)*hypot(f,g); cs=f/radius; sn=g/radius;
            end
            R(j,j)=radius;
            for k=j+1:6
                old=R(j,k); R(j,k)=cs*old+sn*row(k); row(k)=-sn*old+cs*row(k);
            end
            old=rhs(j); rhs(j)=cs*old+sn*u; u=-sn*old+cs*u;
        end
    end
end
valid=abs(diag(R))>eps*10*max(abs(diag(R)));
z=zeros(6,1);
for j=6:-1:1
    if valid(j)
        value=rhs(j);
        for k=j+1:6
            if valid(k), value=value-R(j,k)*z(k); end
        end
        z(j)=value/R(j,j);
    end
end
x=zeros(6,1);
for j=1:6, x(permutation(j))=z(j); end
end

function step=select_step(x,A,g,h,p,ph,d,lb,ub,theta)
if all(x+p>=lb) && all(x+p<=ub), step=p; return; end
[stride,hits]=bound_stride(x,p,lb,ub);
rh=ph; rh(hits)=-rh(hits); reflected=d.*rh;
p=p*stride; ph=ph*stride; on_bound=x+p;
[upper,~]=bound_stride(on_bound,reflected,lb,ub);
lower=(1-theta)*upper; upper=theta*upper;
rvalue=Inf;
if upper>0
    [a,b,c]=line_quadratic(A,g,h,rh,ph);
    [stride,rvalue]=min_line(a,b,c,lower,upper);
    rh=ph+rh*stride; reflected=d.*rh;
end
p=p*theta; ph=ph*theta;
pvalue=quadratic(A,g,ph,h);
agh=-g; ag=d.*agh;
[upper,~]=bound_stride(x,ag,lb,ub); upper=theta*upper;
[a,b,~]=line_quadratic(A,g,h,agh,zeros(6,1));
[stride,agvalue]=min_line(a,b,0,0,upper); ag=ag*stride;
if pvalue<rvalue && pvalue<agvalue, step=p;
elseif rvalue<pvalue && rvalue<agvalue, step=reflected;
else, step=ag;
end
end

function x=reflect(y,lb,ub)
x=y;
if all(y>=lb) && all(y<=ub), return; end
width=ub-lb; z=mod(y-lb,2*width);
x=lb+min(z,2*width-z);
end

function mask=active_bounds(x,lb,ub,tol)
mask=zeros(6,1);
for j=1:6
    if tol==0
        if x(j)<=lb(j), mask(j)=-1; end
        if x(j)>=ub(j), mask(j)=1; end
    else
        lower=x(j)-lb(j); upper=ub(j)-x(j);
        if lower<=min(upper,tol*max(1,abs(lb(j)))), mask(j)=-1; end
        if upper<=min(lower,tol*max(1,abs(ub(j)))), mask(j)=1; end
    end
end
end

function x=interior(x,lb,ub,relative_step)
mask=active_bounds(x,lb,ub,relative_step);
for j=1:6
    if mask(j)==-1
        if relative_step==0, x(j)=lb(j)+eps(lb(j));
        else, x(j)=lb(j)+relative_step*max(1,abs(lb(j))); end
    elseif mask(j)==1
        if relative_step==0, x(j)=ub(j)-eps(ub(j));
        else, x(j)=ub(j)-relative_step*max(1,abs(ub(j))); end
    end
    if x(j)<lb(j) || x(j)>ub(j), x(j)=(lb(j)+ub(j))/2; end
end
end

function [stride,hits]=bound_stride(x,s,lb,ub)
steps=Inf(6,1);
for j=1:6
    if s(j)~=0, steps(j)=max((lb(j)-x(j))/s(j),(ub(j)-x(j))/s(j)); end
end
stride=min(steps); hits=steps==stride;
end

function value=quadratic(A,g,s,h)
v=A*s; value=.5*(v'*v+(s.*h)'*s)+g'*s;
end

function [a,b,c]=line_quadratic(A,g,h,s,s0)
v=A*s; u=A*s0;
a=.5*(v'*v+(s.*h)'*s);
b=g'*s+u'*v+(s0.*h)'*s;
c=.5*(u'*u)+g'*s0+.5*(s0.*h)'*s0;
end

function [t,value]=min_line(a,b,c,lb,ub)
t=lb; value=lb*(a*lb+b)+c;
upper_value=ub*(a*ub+b)+c;
if upper_value<value, t=ub; value=upper_value; end
if a~=0
    stationary=-.5*b/a;
    if stationary>lb && stationary<ub
        stationary_value=stationary*(a*stationary+b)+c;
        if stationary_value<value, t=stationary; value=stationary_value; end
    end
end
end

== matlab function hex_recovery/Task Reference任务参考/Embedded MATLAB ==
  settings: updateMethod=DISCRETE  sampleTime=P.control_dt
  data: t input; observation input; reference output; P_task_reference parameter; audit output
function [reference,audit]=recovery_reference_step(t,observation,P_task_reference)
%#codegen
% Retimes the original geometric path using measured tracking/stability.
% No fault identity, effectiveness, schedule or plant audit is available.
persistent phase progress initialized
if isempty(initialized)
    phase=0; progress=1; initialized=false;
end
r=P_task_reference.control.recovery;
previous=task_reference(phase,P_task_reference);
error=norm(previous(1:3)-observation(1:3));
q=observation(7:10)/norm(observation(7:10));
tilt=acosd(min(max(1-2*(q(1)^2+q(2)^2),-1),1));
rate=norm(observation(11:12));
request=min([ramp(error,r.position_soft_m,r.position_hard_m),...
    ramp(tilt,r.tilt_soft_deg,r.tilt_hard_deg),...
    ramp(rate,r.rate_soft_rad_s,r.rate_hard_rad_s)]);
tau=r.progress_fast_tau_s;
if request<progress, tau=r.progress_slow_tau_s; end
if initialized
    progress=progress+(1-exp(-P_task_reference.control_dt/tau))*(request-progress);
    phase=min(t,phase+P_task_reference.control_dt*progress);
end
reference=task_reference(phase,P_task_reference);
reference(4:6)=progress*reference(4:6);
nominal=task_reference(t,P_task_reference);
audit=[phase;progress;nominal;error;tilt];
initialized=true;
end

function value=ramp(x,soft,hard)
value=min(max((hard-x)/(hard-soft),0),1);
end

function reference=task_reference(t,P_task_reference)
%#codegen
x=P_task_reference.task_origin; v=zeros(3,1);
if P_task_reference.task_family<=3
    u=0; du=0; T=P_task_reference.motion_end-P_task_reference.motion_start;
    if t>=P_task_reference.motion_end
        u=1;
    elseif t>P_task_reference.motion_start
        z=(t-P_task_reference.motion_start)/T;
        u=10*z^3-15*z^4+6*z^5;
        du=30*z^2*(1-z)^2/T;
    end
    if P_task_reference.task_family==1 || P_task_reference.task_family==3
        if P_task_reference.task_family==1
            direction=[cos(P_task_reference.heading);sin(P_task_reference.heading);0];
        else
            direction=[0;0;1];
        end
        delta=P_task_reference.displacement*direction;
        x=x+delta*u; v=delta*du;
    elseif P_task_reference.task_family==2
        angle=P_task_reference.heading+P_task_reference.turn*u; angular_rate=P_task_reference.turn*du;
        radial=[cos(angle);sin(angle);0]; tangent=[-sin(angle);cos(angle);0];
        x=x+P_task_reference.radius*(radial-[cos(P_task_reference.heading);sin(P_task_reference.heading);0]);
        v=P_task_reference.radius*angular_rate*tangent;
    end
elseif P_task_reference.task_family==4
    x=x+[.4*sin(.6*t);.4*(1-cos(.6*t));.15*sin(.4*t)];
    v=[.24*cos(.6*t);.24*sin(.6*t);.06*cos(.4*t)];
elseif P_task_reference.task_family==5 && t>=2
    x=x+[.5;-.4;.3];
elseif P_task_reference.task_family==6 && t>=2 && t<4
    x=x+[0;0;50];
end
reference=[x;v];
end

== matlab function hex_recovery/Fault Injection/Embedded MATLAB ==
  settings: updateMethod=DISCRETE  sampleTime=P.base_dt
  data: t input; segments output; effectiveness output; P_fault_schedule parameter
function [segments,effectiveness]=fault_schedule(t,P_fault_schedule)
%#codegen
% Exact event boundaries, including times between sample ticks.
t=round(t*1e12)/1e12; finish=round((t+P_fault_schedule.base_dt)*1e12)/1e12;
edges=[t;finish;finish;finish]; n=2;
if P_fault_schedule.fault_start>t && P_fault_schedule.fault_start<finish
    n=n+1; edges(n)=P_fault_schedule.fault_start;
end
if P_fault_schedule.fault_end>t && P_fault_schedule.fault_end<finish
    n=n+1; edges(n)=P_fault_schedule.fault_end;
end
edges=sort(edges); segments=zeros(7,3);
effectiveness=eta_at(t,P_fault_schedule);
for i=1:3
    if edges(i+1)>edges(i)
        segments(:,i)=[edges(i+1)-edges(i);eta_at(edges(i),P_fault_schedule)];
    end
end
end

function eta=eta_at(t,P_fault_schedule)
eta=ones(6,1);
if P_fault_schedule.fault_motor>=1 && t>=P_fault_schedule.fault_start && t<P_fault_schedule.fault_end
    eta(P_fault_schedule.fault_motor)=P_fault_schedule.fault_factor;
end
end

== matlab function hex_recovery/Six Rotor Plant/Embedded MATLAB ==
  settings: updateMethod=DISCRETE  sampleTime=P.base_dt
  data: state input; next_state output; command input; segments input; wind input; loads input; P_plant_step parameter
function next_state=plant_step(state,command,segments,wind,loads,P_plant_step)
%#codegen
% RK4 substeps match the original Python event interval partition.
next_state=state;
for j=1:3
    length=segments(1,j);
    if length>0
        count=max(1,ceil(length/P_plant_step.integration_dt-1e-12)); dt=length/count;
        eta=segments(2:7,j);
        for k=1:count
            s=next_state;
            k1=hex_derivative(s,command,eta,wind,loads,P_plant_step);
            k2=hex_derivative(s+dt*k1/2,command,eta,wind,loads,P_plant_step);
            k3=hex_derivative(s+dt*k2/2,command,eta,wind,loads,P_plant_step);
            k4=hex_derivative(s+dt*k3,command,eta,wind,loads,P_plant_step);
            next_state=s+dt*(k1+2*k2+2*k3+k4)/6;
            next_state(7:10)=next_state(7:10)/norm(next_state(7:10));
        end
    end
end
end

function ds=hex_derivative(s,command,eta,wind,loads,P_plant_step)
% Loss acts ONCE on the motor target; actual thrust uses mechanical speed.
R=hex_rotation(s(7:10)); w=s(11:13); omega=s(14:19);
relative=R'*(s(4:6)-wind); force=zeros(3,1); moment=zeros(3,1);
for i=1:6
    r=P_plant_step.rotor_positions(i,:)';
    local=relative+cross(w,r);
    drag=-omega(i)*P_plant_step.rotor_drag.*local;
    thrust=[0;0;P_plant_step.kT(i)*omega(i)^2];
    force=force+thrust+drag;
    moment=moment+cross(r,thrust+drag)+[0;0;P_plant_step.yaw_sign(i)*P_plant_step.kQ(i)*omega(i)^2];
end
force=force-norm(relative)*P_plant_step.body_drag.*relative+loads(1:3);
acceleration=[0;0;-P_plant_step.gravity]+R*force/P_plant_step.mass;
alpha=P_plant_step.invJ*(moment+loads(4:6)-cross(w,P_plant_step.J*w));
ds=[s(4:6);acceleration;.5*hex_multiply(s(7:10),[w;0]);alpha;(sqrt(eta).*command-omega)./P_plant_step.tau];
end

function R=hex_rotation(q)
q=q/norm(q); v=q(1:3); w=q(4);
S=[0 -v(3) v(2);v(3) 0 -v(1);-v(2) v(1) 0];
R=eye(3)+2*w*S+2*S*S;
end

function q=hex_multiply(a,b)
q=[a(4)*b(1:3)+b(4)*a(1:3)+cross(a(1:3),b(1:3));a(4)*b(4)-a(1:3)'*b(1:3)];
end

== matlab function hex_recovery/Sensors and Feedback/Embedded MATLAB ==
  settings: updateMethod=DISCRETE  sampleTime=P.sensor_dt
  data: t input; feedback output; state input; wind input; loads input; observation output; imu output; P_sensor_step parameter
function [feedback,observation,imu]=sensor_step(t,state,wind,loads,P_sensor_step)
%#codegen
% Direct noisy observations, not an estimator. IMU is sensor-frame force/rate.
persistent history samples
if isempty(samples)
    history=zeros(19,1001); samples=0;
end
k=min(size(P_sensor_step.exogenous,1),round(t/P_sensor_step.sensor_dt)+1);
errors=P_sensor_step.exogenous(k,:)';
R=hex_rotation(state(7:10)); w=state(11:13);
ds=hex_derivative(state,zeros(6,1),ones(6,1),wind,loads,P_sensor_step);
r=P_sensor_step.sensor.lever_m; install=P_sensor_step.sensor.installation_matrix;
body=R'*(ds(4:6)+[0;0;P_sensor_step.gravity])+cross(ds(11:13),r)+cross(w,cross(w,r));
accel=install'*body; gyro=install'*w;
observation=state;
if P_sensor_step.noise_enabled
    accel=accel+errors(4:6); gyro=gyro+errors(7:9);
    observation(1:3)=state(1:3)+errors(10:12);
    observation(4:6)=state(4:6)+errors(13:15);
    theta=errors(16:18); angle=norm(theta); dq=[0;0;0;1];
    if angle>1e-14
        dq=[theta*(sin(angle/2)/angle);cos(angle/2)];
    end
    observation(7:10)=hex_multiply(state(7:10),dq);
    observation(7:10)=observation(7:10)/norm(observation(7:10));
    observation(14:19)=state(14:19)+errors(19:24);
end
observation(11:13)=install*gyro;
imu=[accel;gyro];
slot=mod(samples,1001)+1; history(:,slot)=observation; samples=samples+1;
% Latest sensor timestamp <= control timestamp - delay; hold the first sample
% during startup, as the Python history selector does.
delay_ticks=ceil(P_sensor_step.feedback_delay/P_sensor_step.sensor_dt-1e-10);
selected=max(0,samples-1-delay_ticks);
feedback=state;
if P_sensor_step.observed_feedback
    feedback=history(:,mod(selected,1001)+1);
end
end

function ds=hex_derivative(s,command,eta,wind,loads,P_sensor_step)
% Loss acts ONCE on the motor target; actual thrust uses mechanical speed.
R=hex_rotation(s(7:10)); w=s(11:13); omega=s(14:19);
relative=R'*(s(4:6)-wind); force=zeros(3,1); moment=zeros(3,1);
for i=1:6
    r=P_sensor_step.rotor_positions(i,:)';
    local=relative+cross(w,r);
    drag=-omega(i)*P_sensor_step.rotor_drag.*local;
    thrust=[0;0;P_sensor_step.kT(i)*omega(i)^2];
    force=force+thrust+drag;
    moment=moment+cross(r,thrust+drag)+[0;0;P_sensor_step.yaw_sign(i)*P_sensor_step.kQ(i)*omega(i)^2];
end
force=force-norm(relative)*P_sensor_step.body_drag.*relative+loads(1:3);
acceleration=[0;0;-P_sensor_step.gravity]+R*force/P_sensor_step.mass;
alpha=P_sensor_step.invJ*(moment+loads(4:6)-cross(w,P_sensor_step.J*w));
ds=[s(4:6);acceleration;.5*hex_multiply(s(7:10),[w;0]);alpha;(sqrt(eta).*command-omega)./P_sensor_step.tau];
end

function R=hex_rotation(q)
q=q/norm(q); v=q(1:3); w=q(4);
S=[0 -v(3) v(2);v(3) 0 -v(1);-v(2) v(1) 0];
R=eye(3)+2*w*S+2*S*S;
end

function q=hex_multiply(a,b)
q=[a(4)*b(1:3)+b(4)*a(1:3)+cross(a(1:3),b(1:3));a(4)*b(4)-a(1:3)'*b(1:3)];
end

== matlab function hex_recovery/Wind and Body Loads/Embedded MATLAB ==
  settings: updateMethod=DISCRETE  sampleTime=P.sensor_dt
  data: t input; wind output; loads output; P_wind_step parameter
function [wind,loads]=wind_step(t,P_wind_step)
%#codegen
k=min(size(P_wind_step.exogenous,1),round(t/P_wind_step.sensor_dt)+1);
wind=zeros(3,1);
if P_wind_step.wind_enabled
    wind=P_wind_step.exogenous(k,1:3)';
end
loads=[P_wind_step.external_force;P_wind_step.external_torque];
end

== matlab function hex_recovery/Envelope Monitor/Embedded MATLAB ==
  settings: updateMethod=DISCRETE  sampleTime=P.base_dt
  data: state input; stop output; P_envelope_step parameter
function stop=envelope_step(state,P_envelope_step)
%#codegen
b=P_envelope_step.termination;
stop=any(~isfinite(state)) || norm(state(1:3))>b.position_norm_m || ...
    norm(state(4:6))>b.speed_m_s || norm(state(11:13))>b.body_rate_rad_s || state(3)<b.minimum_altitude_m;
end
